simulink model "base_mod"  (Simulink 7.7)
settings: Solver=ode45  StartTime=0.0  StopTime=6.2832  MaxStep=0.062832  RelTol=1e-3
values from neighbouring files (symbols this model uses):
  A = 2    [Base_main.m]    (also in Base_otima_ini.m; Fourier_main.m)
  c = 1    [AMDSB_demodulador_main.m]    (also in AMDSB_nao_linear_main.m; Base_main.m = linspace(0,2,M); base_otima.m = p)
  DC = 50    [Base_main.m]    (also in Base_otima_ini.m; Fourier_main.m)
  n = 1    [Base_main.m]    (also in Base_otima_ini.m; exercicio_01.m = linspace(N_neg,N_pos,N); exercicio_02.m = linspace(N_neg,N_pos,N))
  T = 1.0    (= 1)    [Base_main.m]    (also in Base_otima_ini.m; Fourier_main.m)
undefined symbols (not defined in the file or in its folder): magnitude
settings Model: Creator=vparro  LastModifiedBy=vanderleiparro
settings DebuggingCC: StrictBusMsg=Warning

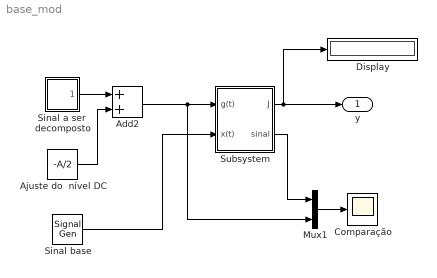
== system base_mod ==
  Add2 : Sum
  Ajuste do  nível DC : Constant  Value=-A/2
  Comparação : Scope
  Display : Display
  Mux1 : Mux  Inputs=2
  Sinal a ser  decomposto : Subsystem  mask(Pulse Generator){period=T, duty=DC, amplitude=A, start=0}
      mask prompts: period "Period (secs):"; duty "Duty cycle (% of period):"; start "Start time:"
      mask help: Pulse Generator
      mask Help: Pulse generator which ensures pulse transitions are hit. Provides a vector of pulses when the height is entered as a vector.  Unmask to see how it works.
      mask Display: plot(0,0,100,100,[95,90,90,75,75,60,60,45,45,30,30,15,15,5],[25,25,75,75,25,25,75,75,25,25,75,75,25,25]);
  Sinal base : SignalGenerator  Frequency=n*inv(T)
  Subsystem : Subsystem
  y : Outport
  wires:
  Sinal a ser  decomposto/1(out1) -> Add2/1
  Ajuste do  nível DC/1 -> Add2/2
  Add2/1 -> Subsystem/1(g(t)), Mux1/2
  Sinal base/1 -> Subsystem/2(x(t))
  Subsystem/1(J) -> y/1, Display/1
  Mux1/1 -> Comparação/1
  Subsystem/2(sinal) -> Mux1/1

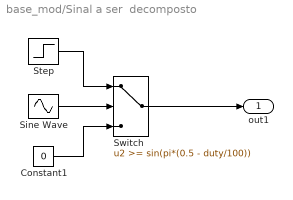
== system base_mod/Sinal a ser  decomposto ==
  Constant1 : Constant  Value=0
  Sine Wave : Sin  Frequency=2*pi./period  Phase=-2*pi*(start./period + duty/200 - 1/4)
  Step : Step  Time=start  After=amplitude
  Switch : Switch  Threshold=sin(pi*(0.5 - duty/100))  SaturateOnIntegerOverflow=on  InputSameDT=on
  out1 : Outport  InitialOutput=0
  wires:
  Step/1 -> Switch/1
  Constant1/1 -> Switch/3
  Switch/1 -> out1/1
  Sine Wave/1 -> Switch/2

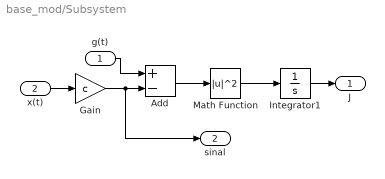
== system base_mod/Subsystem ==
  g(t) : Inport
  x(t) : Inport  Port=2
  Add : Sum  Inputs=+-
  Gain : Gain  Gain=c
  Integrator1 : Integrator
  Math Function : Math  Operator=magnitude^2  SaturateOnIntegerOverflow=on
  J : Outport
  sinal : Outport  Port=2
  wires:
  x(t)/1 -> Gain/1
  Integrator1/1 -> J/1
  g(t)/1 -> Add/1
  Math Function/1 -> Integrator1/1
  Gain/1 -> Add/2, sinal/1
  Add/1 -> Math Function/1
